simulink model "homeMobileManipulator"  (R2026a)
settings: Solver=ode4  StartTime=0  StopTime=Inf  FixedStep=cfg.rates.plant  MaxStep=cfg.rates.plant  AbsTol=1e-8
PostLoadFcn:
  | hmmSetup;
InitFcn:
  | hmmInitializeRun(bdroot);
values from neighbouring files (symbols this model uses):
  armJointLimits = zeros(numel(idx.arm), 2)    [hmmSetup.m]
  cfg = app.RunCfg    [HomeMobileManipulatorApp.m]    (also in HomeMobileManipulatorExample.m = params.cfg; hmmSetup.m = hmmConfig(); setupParams.m = data.cfg)
undefined symbols (not defined in the file or in its folder): actionQueueInit, actorNameTable, Angle, apertureMap, armPlanInit, Axis, basePlanInit, Custom, Extent, gray, gripperCoupling, invalidRayHits, movableRegistry, objectTargetInit, perceptionStatusInit, placeTargetInit, Position, robotStateInit, Sim3dSensor
libraries: robotmaniplib x20, robotcorelib x18, simulink x9, sim3dcameralib x6, sim3dgroundtruthsensorlib x4, dspmtrx3 x3, slpidlib x3, sim3dlib x3, hdlsllib x2, robotsim3dlib x1
(part 5 of 6)

== system homeMobileManipulator/MobileManipulator/Manipulator/MotionPlanning/CandidateIK/Candidate_2/PoseErrCalc ==
  Ta : Inport
  Td : Inport  Port=2
  w : Inport  Port=3
  Angle : Selector  InputPortWidth=4  IndexOptions=Index vector (dialog)  Indices=4  OutputSizes=1
  Axis : Selector  InputPortWidth=4  IndexOptions=Index vector (dialog)  Indices=1:3  OutputSizes=1
  ErrorTform : Product  Inputs=/*  Multiplication=Matrix(*)
  Norm : Sqrt
  OrientWeights : Selector  InputPortWidth=6  IndexOptions=Index vector (dialog)  Indices=1:3  OutputSizes=1
  PosWeights : Selector  InputPortWidth=6  IndexOptions=Index vector (dialog)  Indices=4:6  OutputSizes=1
  RotationVector : Product  Inputs=**
  SumSquares : DotProduct  OutDataTypeStr=Inherit: Inherit via internal rule
  ToAxisAngle : robotcorelib/Coordinate Transformation Conversion  InputRepresentation=Homogeneous Transformation  InputEulerSequence=ZYX  ShowTrVecInputPort=on  OutputRepresentation=Axis-Angle  OutputEulerSequence=ZYX  ShowTrVecOutputPort=on  SimulateUsing=Code generation
  WeightOrient : Product  Inputs=**
  WeightPos : Product  Inputs=**
  WeightedTwist : Concatenate
  poseErrNorm : Outport
  wires:
  Norm/1 -> poseErrNorm/1
  WeightedTwist/1 -> SumSquares/1, SumSquares/2
  WeightOrient/1 -> WeightedTwist/1  "WeightOrient"
  PosWeights/1 -> WeightPos/2
  SumSquares/1 -> Norm/1  "SumSquares"
  OrientWeights/1 -> WeightOrient/2
  RotationVector/1 -> WeightOrient/1  "RotationVector"
  ToAxisAngle/2 -> WeightPos/1
  Angle/1 -> RotationVector/2
  ToAxisAngle/1 -> Axis/1, Angle/1
  Td/1 -> ErrorTform/2
  Axis/1 -> RotationVector/1
  Ta/1 -> ErrorTform/1
  w/1 -> OrientWeights/1, PosWeights/1
  ErrorTform/1 -> ToAxisAngle/1  "ErrorTform"
  WeightPos/1 -> WeightedTwist/2  "WeightPos"

== system homeMobileManipulator/MobileManipulator/Manipulator/MotionPlanning/CandidateIK/Candidate_3/PoseErrCalc ==
  Ta : Inport
  Td : Inport  Port=2
  w : Inport  Port=3
  Angle : Selector  InputPortWidth=4  IndexOptions=Index vector (dialog)  Indices=4  OutputSizes=1
  Axis : Selector  InputPortWidth=4  IndexOptions=Index vector (dialog)  Indices=1:3  OutputSizes=1
  ErrorTform : Product  Inputs=/*  Multiplication=Matrix(*)
  Norm : Sqrt
  OrientWeights : Selector  InputPortWidth=6  IndexOptions=Index vector (dialog)  Indices=1:3  OutputSizes=1
  PosWeights : Selector  InputPortWidth=6  IndexOptions=Index vector (dialog)  Indices=4:6  OutputSizes=1
  RotationVector : Product  Inputs=**
  SumSquares : DotProduct  OutDataTypeStr=Inherit: Inherit via internal rule
  ToAxisAngle : robotcorelib/Coordinate Transformation Conversion  InputRepresentation=Homogeneous Transformation  InputEulerSequence=ZYX  ShowTrVecInputPort=on  OutputRepresentation=Axis-Angle  OutputEulerSequence=ZYX  ShowTrVecOutputPort=on  SimulateUsing=Code generation
  WeightOrient : Product  Inputs=**
  WeightPos : Product  Inputs=**
  WeightedTwist : Concatenate
  poseErrNorm : Outport
  wires:
  Norm/1 -> poseErrNorm/1
  SumSquares/1 -> Norm/1  "SumSquares"
  WeightedTwist/1 -> SumSquares/1, SumSquares/2
  WeightPos/1 -> WeightedTwist/2  "WeightPos"
  WeightOrient/1 -> WeightedTwist/1  "WeightOrient"
  PosWeights/1 -> WeightPos/2
  OrientWeights/1 -> WeightOrient/2
  RotationVector/1 -> WeightOrient/1  "RotationVector"
  Angle/1 -> RotationVector/2
  ToAxisAngle/2 -> WeightPos/1
  ToAxisAngle/1 -> Angle/1, Axis/1
  ErrorTform/1 -> ToAxisAngle/1  "ErrorTform"
  Axis/1 -> RotationVector/1
  Td/1 -> ErrorTform/2
  Ta/1 -> ErrorTform/1
  w/1 -> OrientWeights/1, PosWeights/1

== matlab function homeMobileManipulator/Operator/TaskRequestSource ==
  settings: updateMethod=DISCRETE  sampleTime=cfg.rates.control
  data: task output Bus: TaskRequest
function task = TaskRequestSource()
%TASKREQUESTSOURCE The operator's instruction, as a TaskRequest bus.
%   The model's only task INPUT. It replaced a Constant holding
%   cfg.task.instruction, which was Valid from t = 0 and could never be
%   changed; the sentence is now whatever hmmSubmitTask last submitted, so it
%   can be typed while the model runs and a finished run can be given another
%   one.
%
%   THE FIVE VARIABLES ARE PRE-DECLARED BECAUSE THE CALL IS EXTRINSIC. An
%   extrinsic result is an mxArray until it is assigned into something whose
%   type and size are already known, so these five assignments are what give
%   the outputs their types. They are not defaults for a call that might not
%   happen.
coder.extrinsic('hmmOperatorTask');

codes  = zeros(256, 1, 'uint8');
len    = uint16(0);
taskId = uint32(0);
valid  = false;
cancel = false;

[codes, len, taskId, valid, cancel] = hmmOperatorTask();

task.TaskId         = taskId;
task.Instruction    = codes;
task.InstructionLen = len;
task.SubmitTime     = 0;
task.Cancel         = cancel;
task.Valid          = valid;

== matlab function homeMobileManipulator/Operator/AppStateTap ==
  data: RobotState input Bus: RobotState; TaskResult input Bus: TaskResult; BaseStatus input Bus: BaseStatus; ArmStatus input Bus: ArmStatus; GripperStatus input Bus: GripperStatus; SafetyStatus input Bus: SafetyStatus; ObjectTargetRefined input Bus: ObjectTarget; ObjectTarget input Bus: ObjectTarget; PlaceTarget input Bus: PlaceTarget
function AppStateTap(RobotState, TaskResult, BaseStatus, ArmStatus, GripperStatus, SafetyStatus, ObjectTargetRefined, ObjectTarget, PlaceTarget)
%APPSTATETAP Hand the operator console what it displays (hmmAppStateTap).
%   Display only: nothing in the model reads this block. It runs at a fixed 0.2 s,
%   and does nothing unless HomeMobileManipulatorApp asked for it at Start.
%   SIMULINK-FIRST JUSTIFICATION: publishing to MATLAB appdata for a UI has no block form.
coder.extrinsic('hmmAppStateTap');
hmmAppStateTap(RobotState, TaskResult, BaseStatus, ArmStatus, GripperStatus, SafetyStatus, ObjectTargetRefined, ObjectTarget, PlaceTarget);

== matlab function homeMobileManipulator/Operator/LiveViewTap ==
  data: CameraFrames input; Fired output; LiveViewOn input; StartupOn input boolean
function Fired = LiveViewTap(CameraFrames, LiveViewOn, StartupOn)
%LIVEVIEWTAP Pass each new live-view capture of the four fixed cameras to the operator console.
%   Display only: the frames come from the same CameraRig perception uses, opened for one
%   camera sample every cfg.camera.livePeriod by LiveViewPulse while cfg.camera.liveView is on.
%   A capture is new when camera 1's Timestamp moves; the RGB images then go to
%   hmmLiveViewTap, which stores them for HomeMobileManipulatorApp. Nothing reads Fired.
coder.extrinsic('hmmLiveViewTap');
persistent lastStamp
if isempty(lastStamp)
    lastStamp = -1;
end
Fired = false;
% THE START-UP PICTURE IS PASSED ON WHILE StartupCapture IS OPEN, live view or not - and only
% then, because the frame rendered at t = 0 is dark and must not be the one the console shows.
if (LiveViewOn || StartupOn) && CameraFrames(1).Valid && CameraFrames(1).Timestamp ~= lastStamp
    lastStamp = CameraFrames(1).Timestamp;
    hmmLiveViewTap(CameraFrames(1).RGB, CameraFrames(2).RGB, CameraFrames(3).RGB, ...
        CameraFrames(4).RGB, CameraFrames(1).Timestamp);
    Fired = true;
end

== matlab function homeMobileManipulator/Perception/SceneGrounding/Grounding/GroundingService ==
  data: frames input; ActionQueue output Bus: ActionQueue; task input; requestId input; simTime input; queueTemplate input; Route output; State output; HttpStatus output; Latency output; NumActions output; activeIndex input
function [ActionQueue, Route, State, HttpStatus, Latency, NumActions] = ...
    GroundingService(frames, task, requestId, simTime, queueTemplate, activeIndex)
%#codegen
coder.extrinsic('hmmGroundingService');
ActionQueue = queueTemplate;
Route = uint8(0);
State = uint8(0);
HttpStatus = uint16(0);
Latency = 0;
NumActions = uint8(0);
[ActionQueue, Route, State, HttpStatus, Latency, NumActions] = ...
    hmmGroundingService(frames, task, requestId, simTime, queueTemplate, activeIndex);
end

== matlab function homeMobileManipulator/Perception/SceneGrounding/Reconstruction/TargetReconstruction ==
  data: frames input; obj output Bus: ObjectTarget; queue input; registry input; simTime input; objTemplate input; plcTemplate input; plc output Bus: PlaceTarget
function [obj, plc] = TargetReconstruction(frames, queue, registry, simTime, ...
                                          objTemplate, plcTemplate)
%#codegen
% Gates 6 to 10 and 12: the queue's HEAD action reconstructed to metric 3-D.
% hmmReconstructTargets is extrinsic because it builds a pointCloud and calls
% pcfitplane, both handle-object APIs outside the generated-code subset.
%
% The two templates give the outputs their bus type before the extrinsic call,
% which is the only reason they are arguments. Reconstruction itself is
% MEMORYLESS - the same frames and queue always give the same targets - so the
% templates are ground-value Constants, not the previous answer fed back.
coder.extrinsic('hmmReconstructTargets');

obj = objTemplate;
plc = plcTemplate;

[obj, plc] = hmmReconstructTargets(frames, queue, registry, simTime, ...
    objTemplate, plcTemplate);
end

== matlab function homeMobileManipulator/Perception/SceneGrounding/SceneMapping/MapUpdate ==
  data: frames input; basePose input; grid output; priorGrid input
function grid = MapUpdate(frames, basePose, priorGrid)
%#codegen
% Fold this frame set's calibrated depth returns into the navigation grid.
%
% hmmOccupancyFromDepth is extrinsic because it uses an occupancyMap HANDLE
% object: the log-odds arithmetic, the world-to-grid mapping and the duplicate
% collapse are all inside updateOccupancy, and reimplementing them here to stay
% in the codegen subset would be a second, disagreeing map.
%
% ALL THE MAP STATE IS IN THE DATA STORE, none of it here. priorGrid comes from
% the Data Store Read and the answer goes back to the Data Store Write, so two
% identical calls with the same prior give the same grid.
%
% basePose is passed so the robot's own returns can be discarded - see
% hmmOccupancyFromDepth, THE ROBOT IS NOT AN OBSTACLE TO ITSELF.
coder.extrinsic('hmmOccupancyFromDepth');

grid = priorGrid;
grid = hmmOccupancyFromDepth(frames, basePose, priorGrid);
end

== matlab function homeMobileManipulator/Perception/GraspRefinement/RefineService ==
  data: frames input; RefinedPosition output; task input; coarsePosition input; coarseExtent input; requestId input; simTime input; RefineValid output; RefineStatus output; RefineShift output; ServedRefineId output; RefinedExtent output
function [RefinedPosition, RefineValid, RefineStatus, RefineShift, ServedRefineId, ...
    RefinedExtent] = RefineService(frames, task, coarsePosition, coarseExtent, ...
    requestId, simTime)
%#codegen
% One wrist-refinement transaction. The whole algorithm is hmmRefineService, called
% extrinsically because it reads a file and may open an HTTP connection: nothing in the
% generated-code subset can do either, and the grounding service next door is called the
% same way for the same reason.
%
% EVERY OUTPUT IS GIVEN ITS TYPE BEFORE THE EXTRINSIC CALL. An extrinsic function returns
% an mxArray, which has no Simulink type, so the assignments below are what tell the block
% that RefinedPosition is a 3x1 double, RefineStatus a uint8 and ServedRefineId a uint32.
%
% THE PRE-CALL VALUES ARE ALSO THE SAFE ONES, WHICH IS NOT A COINCIDENCE. RefineValid is
% false here, so if the extrinsic call were removed or failed to assign, ObjectTargetApply
% would pass the coarse point through untouched and the pick would proceed exactly as it
% does with the feature switched off. ServedRefineId stays 0, so the chart would never see
% its request answered and would leave RefineGrasp on tRefineMax instead of hanging.
%
% RefineStatus DEFAULTS TO 1, NOT 0, because 0 is STATUS_APPLIED. A zero default would
% report a successful refinement that never happened; 1 is STATUS_DISABLED, which is the
% honest description of a transaction that did not run.
%
% RefinedExtent DEFAULTS TO THE COARSE EXTENT AND NOT TO ZEROS, which is the one place this
% block's pre-call values are not all-null. RefinedPosition may safely be zeros because
% RefineValid false makes the Switch downstream discard it; the extent takes the same route
% through its own Switch, so the same argument applies - but an extent is also multiplied by
% a grasp clamp and turned into a collision box, and a zeros(3,1) leaking into either would
% be a silent failure rather than a visible one. The coarse extent is the right answer to
% "what if nothing measured anything", so it is what sits here.
%
% THE EXTENT IS AN ARGUMENT BECAUSE THE TWO STAGES RANGE TO DIFFERENT SURFACES, and without
% it the second look would be worse than no second look at all. ObjectTarget.Position is the
% SUPPORT SURFACE beneath the object's centre - that is what a ceiling ray grid whose cells
% are wider than the object itself actually resolves, the cluster being mostly table - while
% the wrist camera, ranging down from the standoff, can only ever reach the object's TOP FACE.
% The two differ by the object's height. hmmWristRefine therefore needs the height twice: to
% convert its measurement back into the field's own units before writing it, and to tell
% "I ranged to the object" apart from "I ranged to the table beside it", which is the one
% failure a close-up refinement is most likely to commit and the one that would otherwise
% move the grasp point down by a full object height while reporting success.
%
% AND IT IS NOW ALSO AN OUTPUT, WHICH IS WHAT CLOSES THE LOOP ON A MEASURED HEIGHT. The same
% frame that locates the top face also measures the support plane under the object, so their
% difference is the object's height, measured - no manifest, no assumption. hmmRefineService
% merges it into element 3 and leaves the horizontal pair alone, and the model's
% MotionPlanning/TargetSelect aims the jaws at hmmGraspAim's clamped mid-height of whatever
% arrives. Without this output the grasp band for an object the scene manifest does not
% describe comes from cfg.percep.extentAssumed, a flat 60 mm guess.
coder.extrinsic('hmmRefineService');

RefinedPosition = zeros(3, 1);
RefineValid     = false;
RefineStatus    = uint8(1);
RefineShift     = 0;
ServedRefineId  = uint32(0);
RefinedExtent   = double(coarseExtent(1:3));

[RefinedPosition, RefineValid, RefineStatus, RefineShift, ServedRefineId, ...
    RefinedExtent] = hmmRefineService(frames, task, coarsePosition, coarseExtent, ...
    requestId, simTime);
end

== matlab function homeMobileManipulator/MobileManipulator/Plant/ChaseViewOn ==
  data: on output boolean
function on = ChaseViewOn()
%CHASEVIEWON Whether the chase camera renders now - see hmmChaseViewOn. Root appdata, read
%   every step, so the app can switch it mid-run: a parameter update cannot (the camera
%   blocks refuse one while running).
coder.extrinsic('hmmChaseViewOn');
on = false;
on = hmmChaseViewOn();

== stateflow chart homeMobileManipulator/TaskPlanner/TaskPlanner ==
  settings: updateMethod=DISCRETE  sampleTime=cfg.rates.supervisor
  state Operating
    en:
    TaskResult.Valid = true;
    TaskResult.Outcome = OUT_PENDING;
    TaskResult.PlannerMode = PL_IDLE;
    TaskResult.TaskId = uint32(0);
    TaskResult.EStopCause = CAUSE_NONE;
    TaskResult.ActiveIndex = uint8(0);
    TaskResult.ActiveVerb = VERB_NONE;
    tTask = Now;
    du:
    TaskResult.Timestamp = Now;
    TaskResult.ElapsedTime = Now - tTask;
    TaskResult.NumActions = qCount;
    TaskResult.NumDone = nDone;
    TaskResult.NumFailed = nFailed;
    TaskResult.ActionState = qExec;
    TaskResult.ActionFailure = qFail;
    TaskResult.Retries = nRetryAction;
    TaskResult.Overflow = qOverflow;
    TaskResult.FailureCode = failCode;
    state Idle
      en:
      TaskResult.PlannerMode = PL_IDLE;
      TaskResult.ActiveIndex = uint8(0);
      TaskResult.ActiveVerb = VERB_NONE;
      RefineRequestId = RefineRequestId + uint32(1);
      PerceptionSend = false;
      RefineSend = false;
      WristCapture = false;
      Cancel = false;
      Stop = false;
      qCount = uint8(0);
      qHead = uint8(0);
      qVerb(:) = uint8(0);
      qExec(:) = uint8(0);
      qFail(:) = uint8(0);
      qOverflow = false;
      nDone = uint8(0);
      nFailed = uint8(0);
      nRetryAction = uint8(0);
      failCode = F_OK;
      tPhase = 0;
      BaseRequest = B_NONE;
      ArmRequest = A_NONE;
      GripRequest = G_NONE;
      du:
      Cancel = false;
      Stop = false;
      tPhase = tPhase + dt;
    state Grounding
      en:
      TaskResult.PlannerMode = PL_GROUND;
      PerceptionSend = true;
      RefineRequestId = RefineRequestId + uint32(1);
      tPhase = 0;
      du:
      PerceptionSend = false;
      tPhase = tPhase + dt;
      ex:
      PerceptionSend = false;
    state Enqueue
      en:
      nNew = ActionQueue.Count;
      qBase = qCount;
      for kIdx = 1:double(nNew)
      if qCount < qCap
      qCount = qCount + uint8(1);
      qVerb(qCount) = ActionQueue.Verb(kIdx);
      qFail(qCount) = ActionQueue.ItemFailure(kIdx);
      if ActionQueue.ItemFailure(kIdx) == F_OK
      qExec(qCount) = EXEC_PENDING;
      else
      qExec(qCount) = EXEC_FAILED;
      nFailed = nFailed + uint8(1);
      end
      else
      qOverflow = true;
      end
      end
      if ActionQueue.Overflow
      qOverflow = true;
      end
      if qOverflow
      failCode = F_QUEUE;
      elseif ActionQueue.FailureCode ~= F_OK
      failCode = ActionQueue.FailureCode;
      end
      if ActionQueue.Head >= uint8(1)
      qHead = qBase + ActionQueue.Head;
      else
      qHead = uint8(0);
      end
    state Dispatch
      en:
      TaskResult.PlannerMode = PL_DISPATCH;
      tPhase = 0;
      RefineRequestId = RefineRequestId + uint32(1);
      if qHead >= uint8(1) && qHead <= qCount
      qExec(qHead) = EXEC_ACTIVE;
      TaskResult.ActiveIndex = qHead;
      TaskResult.ActiveVerb = qVerb(qHead);
      else
      TaskResult.ActiveIndex = uint8(0);
      TaskResult.ActiveVerb = VERB_NONE;
      end
    state NavToPick
      en:
      TaskResult.PlannerMode = PL_NAV_PICK;
      goalPoint = ObjectTarget.Position;
      BaseCarriedExtent = zeroExtent;
      if qVerb(qHead) == VERB_HOME
      BaseGoalPose = [goalPoint(1); goalPoint(2); ObjectTarget.Orientation(1)];
      elseif qVerb(qHead) == VERB_NAVIGATE
      % A MOVE GOES TO THE POINT, NOT A STAND-OFF SHORT OF IT - no arm works from here.
      % BaseGoalSelect keeps it if the base fits, else the nearest pose that does.
      dGoal = goalPoint(1:2) - RobotState.BasePose(1:2);
      BaseGoalPose = [goalPoint(1); goalPoint(2); atan2(dGoal(2), dGoal(1))];
      else
      dGoal = goalPoint(1:2) - RobotState.BasePose(1:2);
      nGoal = max(norm(dGoal), standoffEps);
      BaseGoalPose = [goalPoint(1) - standoff * dGoal(1) / nGoal; goalPoint(2) - standoff * dGoal(2) / nGoal; atan2(dGoal(2), dGoal(1))];
      end
      BaseGoalTarget = goalPoint;
      BaseGoalTolerance = goalTol;
      BaseRequestId = BaseRequestId + uint32(1);
      BaseRequest = B_GOTO;
      tPhase = 0;
      du:
      tPhase = tPhase + dt;
    state Pick
      en:
      TaskResult.PlannerMode = PL_PICK;
      phaseFail = F_OK;
      refineDone = false;
      du:
      tPhase = tPhase + dt;
      state OpenJaws
        en:
        GripRequestId = GripRequestId + uint32(1);
        GripRequest = G_OPEN;
        TargetAperture = aOpen;
        AttachActorId = noneActor;
        tPhase = 0;
        du:
        if GripperStatus.ServedRequestId == GripRequestId && GripperStatus.Mode == M_GRIP_FAULTED
        phaseFail = GripperStatus.FailureCode;
        if phaseFail == F_OK
        phaseFail = F_NOTGRASP;
        end
        elseif tPhase > tGripWait
        phaseFail = F_STALE;
        end
      state PlanPick
        en:
        ArmRequestId = ArmRequestId + uint32(1);
        ArmMode = MODE_PICK;
        ApproachDepth = approachDepth;
        ArmRequest = A_PLAN_PICK;
        tPhase = 0;
        du:
        if ArmStatus.ServedRequestId == ArmRequestId && ArmStatus.State == S_FAILED
        phaseFail = ArmStatus.FailureCode;
        if phaseFail == F_OK
        phaseFail = F_ARM;
        end
        elseif tPhase > tPlanMoveMax
        phaseFail = F_STALE;
        end
      state RefineGrasp
        en:
        RefineRequestId = RefineRequestId + uint32(1);
        RefineSend = true;
        WristCapture = true;
        tPhase = 0;
        du:
        RefineSend = false;
        tPhase = tPhase + dt;
        ex:
        RefineSend = false;
        WristCapture = false;
      state ApproachObject
        en:
        ArmRequestId = ArmRequestId + uint32(1);
        ArmRequest = A_APPROACH;
        tPhase = 0;
        du:
        if ArmStatus.ServedRequestId == ArmRequestId && ArmStatus.State == S_FAILED
        phaseFail = ArmStatus.FailureCode;
        if phaseFail == F_OK
        phaseFail = F_ARM;
        end
        elseif tPhase > tApproachMax
        phaseFail = F_STALE;
        end
      state CloseJaws
        en:
        GripRequestId = GripRequestId + uint32(1);
        GripRequest = G_CLOSE;
        TargetAperture = ArmStatus.ApertureCmd;
        AttachActorId = ArmStatus.AttachActorId;
        tPhase = 0;
        du:
        if GripperStatus.ServedRequestId == GripRequestId && GripperStatus.Mode == M_GRIP_FAULTED
        phaseFail = GripperStatus.FailureCode;
        if phaseFail == F_OK
        phaseFail = F_NOTGRASP;
        end
        elseif tPhase > tGripWait
        phaseFail = F_NOTGRASP;
        end
      state LiftObject
        en:
        ArmRequestId = ArmRequestId + uint32(1);
        ApproachDepth = approachDepth;
        ArmRequest = A_RETREAT;
        tPhase = 0;
        du:
        if ArmStatus.ServedRequestId == ArmRequestId && ArmStatus.State == S_FAILED
        phaseFail = ArmStatus.FailureCode;
        if phaseFail == F_OK
        phaseFail = F_ARM;
        end
        elseif tPhase > tApproachMax
        phaseFail = F_STALE;
        end
      (default) -> OpenJaws
      OpenJaws -> PlanPick : [GripperStatus.ServedRequestId == GripRequestId && ...
          | GripperStatus.Mode == M_GRIP_OPEN && ...
          | GripperStatus.State == S_DONE]
      RefineGrasp -> PlanPick : [ServedRefineId == RefineRequestId || ...
          | tPhase > tRefineMax]
          | {refineDone = true;}
      PlanPick -> RefineGrasp [order 1] : [ArmStatus.ServedRequestId == ArmRequestId && ...
          | ArmStatus.State == S_DONE && ~refineDone]
      PlanPick -> ApproachObject [order 2] : [ArmStatus.ServedRequestId == ArmRequestId && ...
          | ArmStatus.State == S_DONE]
      ApproachObject -> CloseJaws : [ArmStatus.ServedRequestId == ArmRequestId && ...
          | ArmStatus.State == S_DONE]
      CloseJaws -> LiftObject : [GripperStatus.ServedRequestId == GripRequestId && ...
          | GripperStatus.Mode == M_GRIP_VALIDATED]
    state StowLoaded
      en:
      ArmRequestId = ArmRequestId + uint32(1);
      ArmRequest = A_STOW;
      tPhase = 0;
      du:
      if ArmStatus.ServedRequestId == ArmRequestId && ArmStatus.State == S_FAILED
      phaseFail = ArmStatus.FailureCode;
      if phaseFail == F_OK
      phaseFail = F_ARM;
      end
      elseif tPhase > tStowMax
      phaseFail = F_STALE;
      end
    state NavToPlace
      en:
      TaskResult.PlannerMode = PL_NAV_PLACE;
      goalPoint = PlaceTarget.Point;
      BaseCarriedExtent = ObjectTarget.Extent;
      dGoal = goalPoint(1:2) - RobotState.BasePose(1:2);
      nGoal = max(norm(dGoal), standoffEps);
      BaseGoalPose = [goalPoint(1) - standoffPlace * dGoal(1) / nGoal; goalPoint(2) - standoffPlace * dGoal(2) / nGoal; atan2(dGoal(2), dGoal(1))];
      BaseGoalTarget = goalPoint;
      BaseGoalTolerance = goalTol;
      BaseRequestId = BaseRequestId + uint32(1);
      BaseRequest = B_GOTO;
      tPhase = 0;
      du:
      tPhase = tPhase + dt;
    state Place
      en:
      TaskResult.PlannerMode = PL_PLACE;
      phaseFail = F_OK;
      du:
      tPhase = tPhase + dt;
      state PlanPlace
        en:
        ArmRequestId = ArmRequestId + uint32(1);
        ArmMode = MODE_PLACE;
        ApproachDepth = approachDepth;
        ArmRequest = A_PLAN_PLACE;
        tPhase = 0;
        du:
        if ArmStatus.ServedRequestId == ArmRequestId && ArmStatus.State == S_FAILED
        phaseFail = ArmStatus.FailureCode;
        if phaseFail == F_OK
        phaseFail = F_ARM;
        end
        elseif tPhase > tPlanMoveMax
        phaseFail = F_STALE;
        end
      state ApproachSurface
        en:
        ArmRequestId = ArmRequestId + uint32(1);
        ArmRequest = A_APPROACH;
        tPhase = 0;
        du:
        if ArmStatus.ServedRequestId == ArmRequestId && ArmStatus.State == S_FAILED
        phaseFail = ArmStatus.FailureCode;
        if phaseFail == F_OK
        phaseFail = F_ARM;
        end
        elseif tPhase > tApproachMax
        phaseFail = F_STALE;
        end
      state ReleaseJaws
        en:
        GripRequestId = GripRequestId + uint32(1);
        GripRequest = G_OPEN;
        TargetAperture = aOpen;
        AttachActorId = noneActor;
        tPhase = 0;
        du:
        if GripperStatus.ServedRequestId == GripRequestId && GripperStatus.Mode == M_GRIP_FAULTED
        phaseFail = GripperStatus.FailureCode;
        if phaseFail == F_OK
        phaseFail = F_NOTGRASP;
        end
        elseif tPhase > tGripWait
        phaseFail = F_STALE;
        end
      state WithdrawTool
        en:
        ArmRequestId = ArmRequestId + uint32(1);
        ApproachDepth = approachDepth;
        ArmRequest = A_RETREAT;
        tPhase = 0;
        du:
        if ArmStatus.ServedRequestId == ArmRequestId && ArmStatus.State == S_FAILED
        phaseFail = ArmStatus.FailureCode;
        if phaseFail == F_OK
        phaseFail = F_ARM;
        end
        elseif tPhase > tApproachMax
        phaseFail = F_STALE;
        end
      state StowEmpty
        en:
        ArmRequestId = ArmRequestId + uint32(1);
        ArmRequest = A_STOW;
        tPhase = 0;
        du:
        if ArmStatus.ServedRequestId == ArmRequestId && ArmStatus.State == S_FAILED
        phaseFail = ArmStatus.FailureCode;
        if phaseFail == F_OK
        phaseFail = F_ARM;
        end
        elseif tPhase > tStowMax
        phaseFail = F_STALE;
        end
      (default) -> PlanPlace
      PlanPlace -> ApproachSurface : [ArmStatus.ServedRequestId == ArmRequestId && ...
          | ArmStatus.State == S_DONE]
      ApproachSurface -> ReleaseJaws : [ArmStatus.ServedRequestId == ArmRequestId && ...
          | ArmStatus.State == S_DONE]
      ReleaseJaws -> WithdrawTool : [GripperStatus.ServedRequestId == GripRequestId && ...
          | GripperStatus.Mode == M_GRIP_OPEN && ...
          | GripperStatus.State == S_DONE]
      WithdrawTool -> StowEmpty : [ArmStatus.ServedRequestId == ArmRequestId && ...
          | ArmStatus.State == S_DONE]
    state Recover
      en:
      TaskResult.PlannerMode = PL_RECOVER;
      Cancel = true;
      PerceptionSend = false;
      RefineSend = false;
      WristCapture = false;
      BaseRequest = B_NONE;
      ArmRequest = A_NONE;
      GripRequest = G_NONE;
      tPhase = 0;
      du:
      Cancel = false;
      tPhase = tPhase + dt;
    (default) -> Idle
    Idle -> Grounding : [TaskRequest.Valid && ~TaskRequest.Cancel && ...
        | TaskRequest.TaskId ~= taskIdRef]
        | {taskIdRef = TaskRequest.TaskId;
        |  TaskResult.TaskId = TaskRequest.TaskId;
        |  TaskResult.Outcome = OUT_PENDING;
        |  tTask = Now;}
    Recover -> Grounding [order 1] : [tPhase >= tHold && ...
        | nRetryAction < nActionRetry && ...
        | ~RobotState.IsGrasped && ...
        | failCode == F_PLACE_UNREACH && ...
        | nDone == uint8(0)]
        | {nRetryAction = nRetryAction + uint8(1);
        |  qCount = uint8(0);
        |  qHead = uint8(0);
        |  qExec(:) = EXEC_PENDING;
        |  qFail(:) = F_OK;
        |  nFailed = uint8(0);
        |  failCode = F_OK;
        |  groundAfterId = PerceptionStatus.RequestId;
        |  TaskResult.ActiveIndex = uint8(0);
        |  BaseRequest = B_NONE;
        |  ArmRequest = A_NONE;
        |  GripRequest = G_NONE;}
      settings: description=RE-GROUND ON PlaceUnreachable (2026-10-12). The Dispatch retry below excludes code 33 because it reuses the same grounding answer and therefore the same place point. This retry instead asks the provider again: the queue is cleared and TaskResult.ActiveIndex reset to 0, so Grounding takes the fresh-transaction path (hmmGroundingService activeIndex 0) and Enqueue rebuilds the queue from the new answer. A live provider can return a different, serviceable place point - the prompt now steers it towards an open edge; a replay returns the same one and fails as before, one hold later. Bounded by nActionRetry (nRetryAction is not reset by Enqueue), and only while nDone == 0 so no completed action is repeated.
    Recover -> Grounding [order 4] : [tPhase >= tHold && continueOnFail && ...
        | ~RobotState.IsGrasped && ...
        | any(qExec(1:double(qCount)) == EXEC_PENDING)]
        | {qExec(qHead) = EXEC_FAILED;
        |  qFail(qHead) = failCode;
        |  nFailed = nFailed + uint8(1);
        |  qHead = hmmNextPendingAction(qExec, qCount, EXEC_PENDING);
        |  TaskResult.ActiveIndex = qHead;
        |  nRetryAction = uint8(0);
        |  BaseRequest = B_NONE;
        |  ArmRequest = A_NONE;
        |  GripRequest = G_NONE;}
    StowEmpty -> Grounding [order 1] : [ArmStatus.ServedRequestId == ArmRequestId && ...
        | ArmStatus.State == S_DONE && ...
        | any(qExec(1:double(qCount)) == EXEC_PENDING)]
        | {qExec(qHead) = EXEC_DONE;
        |  nDone = nDone + uint8(1);
        |  qHead = hmmNextPendingAction(qExec, qCount, EXEC_PENDING);
        |  TaskResult.ActiveIndex = qHead;
        |  nRetryAction = uint8(0);
        |  BaseRequest = B_NONE;
        |  ArmRequest = A_NONE;
        |  GripRequest = G_NONE;}
    NavToPick -> Grounding [order 2] : [BaseStatus.ServedRequestId == BaseRequestId && ...
        | BaseStatus.State == S_DONE && ...
        | qVerb(qHead) ~= VERB_TRANSFER && ...
        | any(qExec(1:double(qCount)) == EXEC_PENDING)]
        | {qExec(qHead) = EXEC_DONE;
        |  nDone = nDone + uint8(1);
        |  qHead = hmmNextPendingAction(qExec, qCount, EXEC_PENDING);
        |  TaskResult.ActiveIndex = qHead;
        |  nRetryAction = uint8(0);
        |  BaseRequest = B_NONE;
        |  ArmRequest = A_NONE;
        |  GripRequest = G_NONE;}
    Grounding -> Dispatch [order 2] : [TaskResult.ActiveIndex > uint8(0) && ...
        | PerceptionStatus.Valid && ...
        | PerceptionStatus.TaskId == taskIdRef && ...
        | PerceptionStatus.State == PS_COMPLETE && ...
        | ActionQueue.Valid && ...
        | ActionQueue.TaskId == taskIdRef && ...
        | ActionQueue.Head == qHead && ...
        | ActionQueue.RequestId == PerceptionStatus.RequestId]
    Grounding -> Enqueue [order 1] : [TaskResult.ActiveIndex == uint8(0) && ...
        | PerceptionStatus.Valid && ...
        | PerceptionStatus.TaskId == taskIdRef && ...
        | PerceptionStatus.State == PS_COMPLETE && ...
        | ActionQueue.Valid && ...
        | ActionQueue.TaskId == taskIdRef && ...
        | ActionQueue.RequestId == PerceptionStatus.RequestId && ...
        | PerceptionStatus.RequestId > groundAfterId]
    Enqueue -> Dispatch
    Dispatch -> Recover [order 4] : [~ObjectTarget.Valid]
        | {failCode = ObjectTarget.FailureCode;}
    Dispatch -> (junction 207) [order 1] : [(qHead < uint8(1) || qHead > qCount) && ...
        | failCode ~= F_OK]
    Dispatch -> (junction 207) [order 2] : [qHead < uint8(1) || qHead > qCount]
        | {failCode = F_UNKNOWN;}
    Dispatch -> (junction 207) [order 3] : [qVerb(qHead) ~= VERB_TRANSFER && ...
        | qVerb(qHead) ~= VERB_NAVIGATE && ...
        | qVerb(qHead) ~= VERB_HOME]
        | {qExec(qHead) = EXEC_FAILED;
        |  qFail(qHead) = F_UNKNOWN;
        |  nFailed = nFailed + uint8(1);
        |  failCode = F_UNKNOWN;}
    Dispatch -> Recover [order 5] : [qVerb(qHead) == VERB_TRANSFER && ...
        | ~PlaceTarget.Valid]
        | {failCode = PlaceTarget.FailureCode;}
    Recover -> Dispatch [order 2] : [tPhase >= tHold && ...
        | nRetryAction < nActionRetry && ...
        | ~RobotState.IsGrasped && ...
        | failCode ~= F_BASE_START && ...
        | failCode ~= F_BASE_GOAL && ...
        | failCode ~= F_BASE_UNREACH && ...
        | failCode ~= F_PLACE_UNREACH]
        | {nRetryAction = nRetryAction + uint8(1);
        |  qExec(qHead) = EXEC_PENDING;
        |  failCode = F_OK;}
      settings: description=|
          | TWO GUARDS ON THE ACTION RETRY, both of them about attempts that cannot succeed.
          | 
          | ~RobotState.IsGrasped: this transition restarts the WHOLE action at Dispatch, so a transfer restarts at NavToPick and drives back to where the object used to be. If the jaws are holding it, it is not there - it is being carried - so the second grasp cannot succeed and the run ends on a timeout instead of on the failure that happened. Dispatch is the queue's only re-entry, so there is no sound restart point for a half-finished transfer; a failure with the object held is reported, with the object still held.
          | 
          | failCode ~= F_BASE_START / F_BASE_GOAL / F_BASE_UNREACH / F_PLACE_UNREACH: these four are deterministic statements about the map and the pose, and Recover's entry cancels every subordinate so neither changes while it waits. A second identical request returns the identical answer one graspSettle later; all the retries buy is that the phase timeout expires first, so the run reports the timeout instead of the cause it already had. BaseSearchFailed is NOT in the list - BiRRT and RRT* are randomised, so retrying one is a different sample.
          | 
          | F_PLACE_UNREACH is the fourth and it arrives from perception rather than from the base, by way of Dispatch order 5. hmmReconstructTargets raises it on the FIRST perception tick, from the start pose, when no base pose on the stand-off ring can serve the fitted place point - so a restart re-grounds from a pose the base never left, and the second answer is the first. Measured 2026-10-02: the kitchen-counter transfer spent its one retry and reported code 33 at 1.6 s rather than 0.8 s with the identical diagnosis, and the counter's middle scores 0 of 24 free bearings, so there was nothing a second look could have seen. Making that place leg succeed needs candidate place regions ranked by serviceability before one is committed to, which is a different change from this one.
          | 
          | No transition is added: a refused retry falls through to execution orders 2 and 3, which already write qFail(qHead) = failCode.
    Dispatch -> NavToPick [order 6]
    NavToPick -> Recover [order 4] : [tPhase > tNavMax]
        | {failCode = F_PATH;}
    NavToPick -> Recover [order 5] : [BaseStatus.ServedRequestId == BaseRequestId && ...
        | BaseStatus.State == S_FAILED]
        | {failCode = BaseStatus.FailureCode;}
    NavToPick -> Pick [order 1] : [BaseStatus.ServedRequestId == BaseRequestId && ...
        | BaseStatus.State == S_DONE && ...
        | qVerb(qHead) == VERB_TRANSFER]
    LiftObject -> StowLoaded : [ArmStatus.ServedRequestId == ArmRequestId && ...
        | ArmStatus.State == S_DONE]
    StowLoaded -> NavToPlace : [ArmStatus.ServedRequestId == ArmRequestId && ...
        | ArmStatus.State == S_DONE]
    Pick -> Recover : [phaseFail ~= F_OK]
        | {failCode = phaseFail;}
    NavToPlace -> Recover [order 2] : [BaseStatus.ServedRequestId == BaseRequestId && ...
        | BaseStatus.State == S_FAILED]
        | {failCode = BaseStatus.FailureCode;}
    NavToPlace -> Recover [order 3] : [tPhase > tNavMax]
        | {failCode = F_PATH;}
    NavToPlace -> Place [order 1] : [BaseStatus.ServedRequestId == BaseRequestId && ...
        | BaseStatus.State == S_DONE]
    Place -> Recover : [phaseFail ~= F_OK]
        | {failCode = phaseFail;}
  state Failed
    en:
    TaskResult.PlannerMode = PL_FAILED;
    TaskResult.Outcome = OUT_FAILED;
    BaseRequest = B_NONE;
    ArmRequest = A_NONE;
    GripRequest = G_NONE;
    % see this state's Description - a copy of Operating's du, on purpose
    TaskResult.Timestamp = Now;
    TaskResult.ElapsedTime = Now - tTask;
    TaskResult.NumActions = qCount;
    TaskResult.NumDone = nDone;
    TaskResult.NumFailed = nFailed;
    TaskResult.ActionState = qExec;
    TaskResult.ActionFailure = qFail;
    TaskResult.Retries = nRetryAction;
    TaskResult.Overflow = qOverflow;
    TaskResult.FailureCode = failCode;
    settings: description=|
        | THE TEN TaskResult PUBLICATION LINES IN THIS ENTRY ACTION ARE A COPY OF Operating's du
        | ACTION. CHANGE ONE AND CHANGE ALL FOUR SITES - Operating (du), Done, Failed, Stopped.
        | 
        | Why they have to be here at all. The task-result counters are incremented in TRANSITION
        | actions on the transitions that LEAVE Operating: NavToPick -> Done and
        | Place/StowEmpty -> Done write qExec(qHead) = EXEC_DONE and nDone++, while
        | Recover -> Done and Recover -> Failed write qExec = EXEC_FAILED, qFail(qHead) = failCode
        | and nFailed++. Stateflow evaluates a state's outgoing transitions BEFORE its during
        | action, so on the tick one of those fires, Operating's du has ALREADY run for that step -
        | and Operating is then inactive, so it never runs again. The last values Operating
        | published are therefore always the PRE-INCREMENT ones and no later tick can correct them.
        | 
        | Measured on a failed run: Outcome 3 and FailureCode 27 were
        | both correct, because Done's entry and failCode are inside Operating, while NumFailed
        | read 0 instead of 1, ActionFailure was all-zero in every sample instead of 27 at qHead,
        | ActionState stayed pinned at EXEC_ACTIVE from 0.5 s to the end instead of EXEC_FAILED,
        | and ElapsedTime froze at 18.34 s on a run that reached 18.98 s. Three independently wrong
        | fields, five writes from one transition, one cause. And on every SUCCESS run,
        | TaskResult.NumDone read 0 beside an Outcome of OUT_SUCCESS - the mismatch that made this
        | look like a counting bug for months. It is not: Done's entry reads nDone = 1 to DECIDE
        | OUT_SUCCESS and then left the stale 0 published next to it.
        | 
        | Stopped already carried two of these ten lines - Timestamp and ElapsedTime - which means
        | the E-stop path was patched for exactly this defect and the other eight were missed. That
        | drift is the argument for a single publishTaskResult() function called from all four
        | sites, which is the structurally correct fix and is NOT what is here: this chart has no
        | graphical, MATLAB or truth-table functions, and adding the first one is a larger change
        | than the defect warrants. If a fifth site ever
        | needs these lines, build the function instead of copying them again.
  state Stopped
    en:
    TaskResult.PlannerMode = PL_STOPPED;
    TaskResult.Outcome = OUT_ABORTED;
    TaskResult.EStopCause = SafetyStatus.Cause;
    Stop = true;
    Cancel = false;
    PerceptionSend = false;
    RefineSend = false;
    WristCapture = false;
    BaseRequest = B_NONE;
    ArmRequest = A_NONE;
    GripRequest = G_NONE;
    % see this state's Description - a copy of Operating's du, on purpose
    TaskResult.Timestamp = Now;
    TaskResult.ElapsedTime = Now - tTask;
    TaskResult.NumActions = qCount;
    TaskResult.NumDone = nDone;
    TaskResult.NumFailed = nFailed;
    TaskResult.ActionState = qExec;
    TaskResult.ActionFailure = qFail;
    TaskResult.Retries = nRetryAction;
    TaskResult.Overflow = qOverflow;
    TaskResult.FailureCode = failCode;
    settings: description=|
        | THE TEN TaskResult PUBLICATION LINES IN THIS ENTRY ACTION ARE A COPY OF Operating's du
        | ACTION. CHANGE ONE AND CHANGE ALL FOUR SITES - Operating (du), Done, Failed, Stopped.
        | 
        | Why they have to be here at all. The task-result counters are incremented in TRANSITION
        | actions on the transitions that LEAVE Operating: NavToPick -> Done and
        | Place/StowEmpty -> Done write qExec(qHead) = EXEC_DONE and nDone++, while
        | Recover -> Done and Recover -> Failed write qExec = EXEC_FAILED, qFail(qHead) = failCode
        | and nFailed++. Stateflow evaluates a state's outgoing transitions BEFORE its during
        | action, so on the tick one of those fires, Operating's du has ALREADY run for that step -
        | and Operating is then inactive, so it never runs again. The last values Operating
        | published are therefore always the PRE-INCREMENT ones and no later tick can correct them.
        | 
        | Measured on a failed run: Outcome 3 and FailureCode 27 were
        | both correct, because Done's entry and failCode are inside Operating, while NumFailed
        | read 0 instead of 1, ActionFailure was all-zero in every sample instead of 27 at qHead,
        | ActionState stayed pinned at EXEC_ACTIVE from 0.5 s to the end instead of EXEC_FAILED,
        | and ElapsedTime froze at 18.34 s on a run that reached 18.98 s. Three independently wrong
        | fields, five writes from one transition, one cause. And on every SUCCESS run,
        | TaskResult.NumDone read 0 beside an Outcome of OUT_SUCCESS - the mismatch that made this
        | look like a counting bug for months. It is not: Done's entry reads nDone = 1 to DECIDE
        | OUT_SUCCESS and then left the stale 0 published next to it.
        | 
        | Stopped already carried two of these ten lines - Timestamp and ElapsedTime - which means
        | the E-stop path was patched for exactly this defect and the other eight were missed. That
        | drift is the argument for a single publishTaskResult() function called from all four
        | sites, which is the structurally correct fix and is NOT what is here: this chart has no
        | graphical, MATLAB or truth-table functions, and adding the first one is a larger change
        | than the defect warrants. If a fifth site ever
        | needs these lines, build the function instead of copying them again.
  state Cancelled
    en:
    TaskResult.PlannerMode = PL_IDLE;
    TaskResult.Outcome = OUT_ABORTED;
    TaskResult.EStopCause = CAUSE_NONE;
    Stop = false;
    Cancel = true;
    PerceptionSend = false;
    RefineSend = false;
    WristCapture = false;
    BaseRequest = B_NONE;
    ArmRequest = A_NONE;
    GripRequest = G_NONE;
    % see this state's Description - a copy of Operating's du, on purpose
    TaskResult.Timestamp = Now;
    TaskResult.ElapsedTime = Now - tTask;
    TaskResult.NumActions = qCount;
    TaskResult.NumDone = nDone;
    TaskResult.NumFailed = nFailed;
    TaskResult.ActionState = qExec;
    TaskResult.ActionFailure = qFail;
    TaskResult.Retries = nRetryAction;
    TaskResult.Overflow = qOverflow;
    TaskResult.FailureCode = failCode;
  state Done
    en:
    TaskResult.PlannerMode = PL_DONE;
    nAdmissible = uint8(0);
    for kIdx = 1:double(qCount)
    if qFail(kIdx) == F_OK
    nAdmissible = nAdmissible + uint8(1);
    end
    end
    if nDone == uint8(0)
    TaskResult.Outcome = OUT_FAILED;
    elseif nFailed > uint8(0) || nDone < nAdmissible || qOverflow
    TaskResult.Outcome = OUT_PARTIAL;
    else
    TaskResult.Outcome = OUT_SUCCESS;
    end
    BaseRequest = B_NONE;
    ArmRequest = A_NONE;
    GripRequest = G_NONE;
    % see this state's Description - a copy of Operating's du, on purpose
    TaskResult.Timestamp = Now;
    TaskResult.ElapsedTime = Now - tTask;
    TaskResult.NumActions = qCount;
    TaskResult.NumDone = nDone;
    TaskResult.NumFailed = nFailed;
    TaskResult.ActionState = qExec;
    TaskResult.ActionFailure = qFail;
    TaskResult.Retries = nRetryAction;
    TaskResult.Overflow = qOverflow;
    TaskResult.FailureCode = failCode;
    settings: description=|
        | THE TEN TaskResult PUBLICATION LINES IN THIS ENTRY ACTION ARE A COPY OF Operating's du
        | ACTION. CHANGE ONE AND CHANGE ALL FOUR SITES - Operating (du), Done, Failed, Stopped.
        | 
        | Why they have to be here at all. The task-result counters are incremented in TRANSITION
        | actions on the transitions that LEAVE Operating: NavToPick -> Done and
        | Place/StowEmpty -> Done write qExec(qHead) = EXEC_DONE and nDone++, while
        | Recover -> Done and Recover -> Failed write qExec = EXEC_FAILED, qFail(qHead) = failCode
        | and nFailed++. Stateflow evaluates a state's outgoing transitions BEFORE its during
        | action, so on the tick one of those fires, Operating's du has ALREADY run for that step -
        | and Operating is then inactive, so it never runs again. The last values Operating
        | published are therefore always the PRE-INCREMENT ones and no later tick can correct them.
        | 
        | Measured on a failed run: Outcome 3 and FailureCode 27 were
        | both correct, because Done's entry and failCode are inside Operating, while NumFailed
        | read 0 instead of 1, ActionFailure was all-zero in every sample instead of 27 at qHead,
        | ActionState stayed pinned at EXEC_ACTIVE from 0.5 s to the end instead of EXEC_FAILED,
        | and ElapsedTime froze at 18.34 s on a run that reached 18.98 s. Three independently wrong
        | fields, five writes from one transition, one cause. And on every SUCCESS run,
        | TaskResult.NumDone read 0 beside an Outcome of OUT_SUCCESS - the mismatch that made this
        | look like a counting bug for months. It is not: Done's entry reads nDone = 1 to DECIDE
        | OUT_SUCCESS and then left the stale 0 published next to it.
        | 
        | Stopped already carried two of these ten lines - Timestamp and ElapsedTime - which means
        | the E-stop path was patched for exactly this defect and the other eight were missed. That
        | drift is the argument for a single publishTaskResult() function called from all four
        | sites, which is the structurally correct fix and is NOT what is here: this chart has no
        | graphical, MATLAB or truth-table functions, and adding the first one is a larger change
        | than the defect warrants. If a fifth site ever
        | needs these lines, build the function instead of copying them again.
  (default) -> Operating
  Cancelled -> Idle : [TaskRequest.Valid && ~TaskRequest.Cancel && ...
      | TaskRequest.TaskId ~= taskIdRef]
  Done -> Idle : [TaskRequest.Valid && ~TaskRequest.Cancel && ...
      | TaskRequest.TaskId ~= taskIdRef]
  Failed -> Idle : [TaskRequest.Valid && ~TaskRequest.Cancel && ...
      | TaskRequest.TaskId ~= taskIdRef]
  (junction 207) -> Failed
  Grounding -> Failed [order 3] : [tPhase > tGroundMax]
      | {failCode = F_PROV_TIMEOUT;}
  Grounding -> Failed [order 4] : [PerceptionStatus.Valid && ...
      | PerceptionStatus.TaskId == taskIdRef && ...
      | PerceptionStatus.State == PS_FAILED]
      | {failCode = PerceptionStatus.FailureCode;}
  Recover -> Failed [order 3] : [tPhase >= tHold && ...
      | (~continueOnFail || RobotState.IsGrasped)]
      | {qExec(qHead) = EXEC_FAILED;
      |  qFail(qHead) = failCode;
      |  nFailed = nFailed + uint8(1);}
  NavToPick -> Done [order 3] : [BaseStatus.ServedRequestId == BaseRequestId && ...
      | BaseStatus.State == S_DONE && ...
      | qVerb(qHead) ~= VERB_TRANSFER && ...
      | ~any(qExec(1:double(qCount)) == EXEC_PENDING)]
      | {qExec(qHead) = EXEC_DONE;
      |  nDone = nDone + uint8(1);}
  Operating -> Stopped [order 1] : [SafetyStatus.EStop]
  Operating -> Cancelled [order 2] : [TaskRequest.Cancel && ...
      | TaskRequest.TaskId == taskIdRef && ...
      | ~in(Operating.Idle)]
  Recover -> Done [order 5] : [tPhase >= tHold && ...
      | ~any(qExec(1:double(qCount)) == EXEC_PENDING)]
      | {qExec(qHead) = EXEC_FAILED;
      |  qFail(qHead) = failCode;
      |  nFailed = nFailed + uint8(1);}
  StowEmpty -> Done [order 2] : [ArmStatus.ServedRequestId == ArmRequestId && ...
      | ArmStatus.State == S_DONE && ...
      | ~any(qExec(1:double(qCount)) == EXEC_PENDING)]
      | {qExec(qHead) = EXEC_DONE;
      |  nDone = nDone + uint8(1);}
  data: TaskRequest input Bus: TaskRequest; ActionQueue input Bus: ActionQueue; PerceptionStatus input Bus: PerceptionStatus; ObjectTarget input Bus: ObjectTarget; PlaceTarget input Bus: PlaceTarget; RobotState input Bus: RobotState; BaseStatus input Bus: BaseStatus; ArmStatus input Bus: ArmStatus; GripperStatus input Bus: GripperStatus; SafetyStatus input Bus: SafetyStatus; Now input double; PerceptionSend output boolean =0; BaseRequest output uint8 =0; BaseRequestId output uint32 =0; BaseGoalPose output double size=[3 1] =0; BaseGoalTarget output double size=[3 1]; BaseGoalTolerance output double size=[3 1] =cfg.plan.baseGoalTolerance(:); BaseCarriedExtent output double size=[3 1] =0; ArmRequest output uint8 =0; ArmRequestId output uint32 =0; ArmMode output uint8 =cfg.plan.ARM_MODE_PICK; ApproachDepth output double =cfg.sup.approachDepth; GripRequest output uint8 =0; GripRequestId output uint32 =0; TargetAperture output double =cfg.gripper.maxOpenPos; AttachActorId output uint8 =cfg.actor.noneId; Cancel output boolean =0; Stop output boolean =0; TaskResult output Bus: TaskResult size=1 =taskResultInit; qCount local uint8 =0; qHead local uint8 =0; qVerb local uint8 size=[8 1] =0; qExec local uint8 size=[8 1] =0; qFail local uint8 size=[8 1] =0; qOverflow local boolean =0; taskIdRef local uint32 =0; tPhase local double =0; tTask local double =0; nRetryAction local uint8 =0; nDone local uint8 =0; nFailed local uint8 =0; failCode local uint8 =0; goalPoint local double size=[3 1] =0; dGoal local double size=[2 1] =0; nGoal local double =0; dt constant double =cfg.rates.supervisor; qCap constant uint8 =cfg.queue.capacity; VERB_TRANSFER constant uint8 =cfg.queue.VERB_TRANSFER; VERB_NAVIGATE constant uint8 =cfg.queue.VERB_NAVIGATE; EXEC_PENDING constant uint8 =cfg.queue.EXEC_PENDING; EXEC_ACTIVE constant uint8 =cfg.queue.EXEC_ACTIVE; EXEC_DONE constant uint8 =cfg.queue.EXEC_DONE; EXEC_FAILED constant uint8 =cfg.queue.EXEC_FAILED; PL_IDLE constant uint8 =cfg.sup.pl.IDLE; PL_GROUND constant uint8 =cfg.sup.pl.GROUND; PL_DISPATCH constant uint8 =cfg.sup.pl.DISPATCH; PL_NAV_PICK constant uint8 =cfg.sup.pl.NAV_TO_PICK; PL_PICK constant uint8 =cfg.sup.pl.PICK; PL_NAV_PLACE constant uint8 =cfg.sup.pl.NAV_TO_PLACE; PL_PLACE constant uint8 =cfg.sup.pl.PLACE; PL_RECOVER constant uint8 =cfg.sup.pl.RECOVER; PL_DONE constant uint8 =cfg.sup.pl.DONE; PL_FAILED constant uint8 =cfg.sup.pl.FAILED; PL_STOPPED constant uint8 =cfg.sup.pl.STOPPED; OUT_PENDING constant uint8 =cfg.sup.out.PENDING; OUT_SUCCESS constant uint8 =cfg.sup.out.SUCCESS; OUT_PARTIAL constant uint8 =cfg.sup.out.PARTIAL; OUT_FAILED constant uint8 =cfg.sup.out.FAILED; OUT_ABORTED constant uint8 =cfg.sup.out.ABORTED; S_DONE constant uint8 =cfg.sup.st.DONE; S_FAILED constant uint8 =cfg.sup.st.FAILED; B_NONE constant uint8 =cfg.sup.baseReq.NONE; B_GOTO constant uint8 =cfg.sup.baseReq.GOTO; A_NONE constant uint8 =cfg.sup.armReq.NONE; A_PLAN_PICK constant uint8 =cfg.sup.armReq.PLAN_PICK; A_PLAN_PLACE constant uint8 =cfg.sup.armReq.PLAN_PLACE; A_APPROACH constant uint8 =cfg.sup.armReq.APPROACH; A_RETREAT constant uint8 =cfg.sup.armReq.RETREAT; A_STOW constant uint8 =cfg.sup.armReq.STOW; G_NONE constant uint8 =cfg.sup.gripReq.NONE; G_OPEN constant uint8 =cfg.sup.gripReq.OPEN; G_CLOSE constant uint8 =cfg.sup.gripReq.CLOSE; M_GRIP_OPEN constant uint8 =cfg.sup.grip.OPEN; M_GRIP_VALIDATED constant uint8 =cfg.sup.grip.VALIDATED; M_GRIP_FAULTED constant uint8 =cfg.sup.grip.FAULTED; F_OK constant uint8 =cfg.fail.OK; F_UNKNOWN constant uint8 =cfg.fail.UnknownAction; F_PROV_TIMEOUT constant uint8 =cfg.fail.ProviderTimeout; F_QUEUE constant uint8 =cfg.fail.QueueOverflow; F_PATH constant uint8 =cfg.fail.PathPlanFailed; F_ARM constant uint8 =cfg.fail.ArmPlanFailed; F_NOTGRASP constant uint8 =cfg.fail.NotGraspable; PS_COMPLETE constant uint8 =uint8(2); PS_FAILED constant uint8 =uint8(3); MODE_PICK constant uint8 =cfg.plan.ARM_MODE_PICK; MODE_PLACE constant uint8 =cfg.plan.ARM_MODE_PLACE; tGroundMax constant double =cfg.sup.timeout.ground; tNavMax constant double =cfg.sup.retry.basePlan * cfg.sup.timeout.basePlan + cfg.sup.timeout.follow; tPlanMoveMax constant double =cfg.sup.retry.armPlan * cfg.sup.timeout.armPlan + cfg.sup.timeout.armMove; tApproachMax constant double =cfg.sup.timeout.approach; tStowMax constant double =cfg.sup.timeout.stow; tGripWait constant double =3 * cfg.sup.timeout.grip; tHold constant double =cfg.sup.graspSettle; nActionRetry constant uint8 =cfg.sup.retry.action; continueOnFail constant boolean =cfg.sup.continueOnActionFailure; standoff constant double =cfg.sup.baseStandoff; standoffEps constant double =0.1 * cfg.sup.baseStandoff; approachDepth constant double =cfg.sup.approachDepth; goalTol constant double size=[3 1] =cfg.plan.baseGoalTolerance(:); zeroExtent constant double size=[3 1] =zeros(3, 1); aOpen constant double =cfg.gripper.maxOpenPos; noneActor constant uint8 =cfg.actor.noneId; kIdx local double =0; nNew local uint8 =0; qBase local uint8 =0; nAdmissible local uint8 =0; VERB_NONE constant uint8 =cfg.queue.VERB_NONE; CAUSE_NONE constant uint8 =cfg.sup.cause.NONE; phaseFail local uint8 =0; F_STALE constant uint8 =cfg.fail.Stale; standoffPlace constant double =cfg.sup.placeStandoff; VERB_HOME constant uint8 =cfg.queue.VERB_HOME; F_BASE_START constant uint8 =cfg.fail.BaseStartOccupied; F_BASE_GOAL constant uint8 =cfg.fail.BaseGoalOccupied; F_BASE_UNREACH constant uint8 =cfg.fail.BaseGoalUnreachable; RefineSend output boolean =0; WristCapture output boolean =0; RefineRequestId output uint32 =0; ServedRefineId input uint32; refineDone local boolean =0; tRefineMax constant double =cfg.sup.timeout.refine; F_PLACE_UNREACH constant uint8 =cfg.fail.PlaceUnreachable; groundAfterId local uint32 =0
  data groundAfterId settings: description=PerceptionStatus.RequestId at a PlaceUnreachable re-ground; Grounding -> Enqueue waits for a newer answer, because the old one still matches the task.

== matlab function homeMobileManipulator/TaskPlanner/BaseGoalSelect ==
  data: gridMatrix input; goalPose output; goalIn input; target input; carriedExtent input; altGoalPose output
function [goalPose, altGoalPose] = BaseGoalSelect(gridMatrix, goalIn, target, carriedExtent)
%#codegen
% Rotate the chart's stand-off onto a bearing the occupancy map says is free.
%
% hmmSelectBaseGoal is extrinsic for the same reasons hmmPlanBasePath is: every
% object it needs - occupancyMap, stateSpaceSE2, validatorOccupancyMap - is a handle
% object with no block form, and the bearing search runs a data-dependent number of
% validity checks, which a fixed block diagram cannot express.
%
% target IS PUBLISHED BY THE CHART RATHER THAN INFERRED HERE. The stand-off can only
% be rotated about the point it was measured from, and while that point is recoverable
% from goalIn alone - the goal is the target pushed back along the goal's own yaw -
% recovering it that way would weld this block to the arithmetic of two Stateflow
% state actions, silently, with nothing to fail if either changed.
%
% THE GOAL PASSES THROUGH UNCHANGED IN TWO CASES AND BOTH MATTER: when the chart's own
% bearing is already free, so a run that never needed this is bit-identical, and when
% NO bearing is free, which is what keeps hmmPlanBasePath's BaseGoalOccupied reachable.
% This block improves a goal or leaves it alone; it cannot manufacture success.
%
% altGoalPose IS AN OFFER, NOT A DECISION: the same position at a roughly opposite heading
% that passes the same footprint and arm-reach screen (hmmStandoffPartner), or goalPose itself
% when none does. MobileBase/PathPlanning plans both and keeps the cheaper drive.
coder.extrinsic('hmmSelectBaseGoal');

goalPose = goalIn;
altGoalPose = goalIn;
[goalPose, ~, ~, altGoalPose] = hmmSelectBaseGoal(gridMatrix, goalIn, target, carriedExtent);
end
